simulink model "task1_oscillator"  (R2023a)
settings: Solver=ode45  StartTime=0  StopTime=30  RelTol=1e-6  AbsTol=1e-9
InitFcn:
  | m=1; k=0.5; l=4; x0=1; v0=0;
Description:
  | Zadanie 1: m x''+k x'+l x=0; x=u[1], v=x'=u[2]. k=0 garmonich., 0<k<2*sqrt(l/m) zatuhanie, k>2*sqrt(l/m) aperiodich.
settings Model: Creator=maybn  LastModifiedBy=maybn
settings OptimizationCC: BlockReduction=off  BooleanDataType=off
settings DebuggingCC: SaveWithParameterizedLinksMsg=none  UnderspecifiedInitializationDetection=Classic  MergeDetectMultiDrivingBlocksExec=none  SignalResolutionControl=TryResolveAllWithWarning
settings HardwareCC: TargetUnknown=on
settings ModelReferenceCC: PropagateSignalLabelsOutOfModel=off

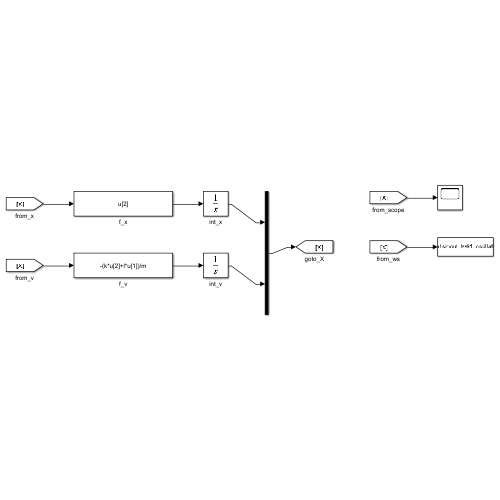
[thumbnail: Simulink's stored preview of the top-level diagram]
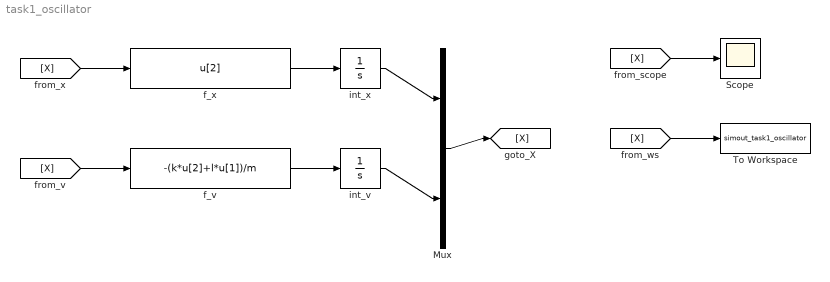
== system task1_oscillator ==
  Mux : Mux  Inputs=2
  Scope : Scope
  To Workspace : ToWorkspace  VariableName=simout_task1_oscillator
  f_v : Fcn  Expr=-(k*u[2]+l*u[1])/m
  f_x : Fcn  Expr=u[2]
  int_v : Integrator  InitialCondition=v0
  int_x : Integrator  InitialCondition=x0
  wires:
  [X] -> f_x/1
  f_x/1 -> int_x/1
  int_x/1 -> Mux/1
  [X] -> f_v/1
  f_v/1 -> int_v/1
  int_v/1 -> Mux/2
  Mux/1 -> [X]
  [X] -> Scope/1
  [X] -> To Workspace/1
